simulink model "Non_linear_simulation_r2018b"  (R2026a)
settings: Solver=ode45  StopTime=5  FixedStep=.002  EnableMultiTasking=on
values from neighbouring files (symbols this model uses):
  A_obs = A - L*C    [MA6217_intial.m]    (also in oberver_performance.m; step1.m = A-L*C)
  alphaPlotHandle = plot(inf,inf,'-b','linewidth',2)    [initialiseVisualiser.m]
  armPartPatchHandle = patch(Xt,Yt,Zt,C,'Edgecolor', edgecolor,'facealpha',facealpha,'clipping','off')    [initialiseVisualiser.m]
  armPartVertices = [X(:) Y(:) Z(:) ones(length(X(:)),1)]'    [initialiseVisualiser.m]
  B_obs = [B, L]    [MA6217_intial.m]    (also in oberver_performance.m = [B L]; step1.m = [B L])
  Bp = 0.0024    [AAP5_setup.m]    (also in plant_parameters.m)
  Br = 0.0024    [AAP5_setup.m]    (also in plant_parameters.m)
  C_obs = eye(4)    [MA6217_intial.m]    (also in oberver_performance.m; step1.m)
  D_obs = zeros(4,3)    [MA6217_intial.m]    (also in oberver_performance.m; step1.m)
  drivePartPatchHandle = patch(Xt,Yt,Zt,C,'Edgecolor', edgecolor,'facealpha',facealpha,'clipping','off')    [initialiseVisualiser.m]
  drivePartVertices = [X(:) Y(:) Z(:) ones(length(X(:)),1)]'    [initialiseVisualiser.m]
  eta_g = 0.9    [AAP5_setup.m]    (also in plant_parameters.m)
  eta_m = 0.69    [AAP5_setup.m]    (also in plant_parameters.m)
  frameRate = 50    [AAP5_setup.m]
  G = N4/N5 * N2/N3    (= 70)    [AAP5_setup.m]    (also in oberver_performance.m = [0 0; plant_parameters.m)
  g = 9.81    [AAP5_setup.m]    (also in plant_parameters.m)
  J = Jarm + Jrotor_eff    (= 0.00608016405667)    [AAP5_setup.m]    (also in plant_parameters.m)
  Jp = mp*Lp^2/12    (= 0.00119873080146)    [AAP5_setup.m]    (also in plant_parameters.m)
  K = K_all(selected_case,:)    [lqr_design.m]    (also in step2.m; step3.m = baseline.K; verify_feedforward.m = design.Kx)
  kb = kt    (= 0.00768)    [AAP5_setup.m]    (also in plant_parameters.m)
  kt = 7.68e-3    (= 0.00768)    [AAP5_setup.m]    (also in plant_parameters.m)
  Lp = 0.33655    [AAP5_setup.m]    (also in plant_parameters.m)
  lp = Lp/2    (= 0.168275)    [AAP5_setup.m]    (also in plant_parameters.m)
  mp = 0.127    [AAP5_setup.m]    (also in plant_parameters.m)
  pendPartPatchHandle = patch(Xt,Yt,Zt,C,'Edgecolor', edgecolor,'facealpha',facealpha,'clipping','off')    [initialiseVisualiser.m]
  pendPartVertices = [X(:) Y(:) Z(:) ones(length(X(:)),1)]'    [initialiseVisualiser.m]
  r = 0.2159    [AAP5_setup.m]    (also in plant_parameters.m)
  Ra = 2.6    [AAP5_setup.m]    (also in plant_parameters.m)
  thetaPlotHandle = plot(inf,inf,'-r','linewidth',2)    [initialiseVisualiser.m]
  x0 = [0; deg2rad(5); 0; 0]    [lqr_design.m]    (also in step2.m = [0; 5*pi/180; 0; 0])
settings Model: Creator=Dylan  LastModifiedBy=DELL
settings DataIOCC: SaveFormat=StructureWithTime
settings HardwareCC: ProdHWDeviceType=Specified

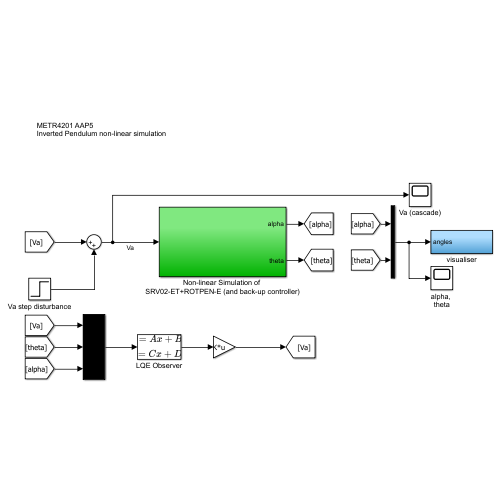
[thumbnail: Simulink's stored preview of the top-level diagram]
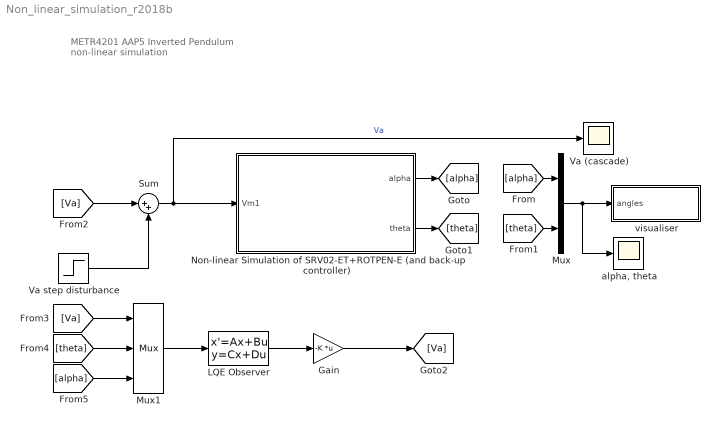
== system Non_linear_simulation_r2018b ==
  note: METR4201 AAP5
      | Inverted Pendulum non-linear simulation
  Gain : Gain  Gain=-K  Multiplication=Matrix(K*u)
  LQE Observer : StateSpace  A=A_obs  B=B_obs  C=C_obs  D=D_obs  InitialCondition=x0
  Mux : Mux  Inputs=2
  Mux1 : Mux  Inputs=3
  Non-linear Simulation of SRV02-ET+ROTPEN-E (and back-up controller) : Subsystem
  Sum : Sum  Inputs=|++
  Va (cascade) : Scope
      settings: ActiveDisplayYMinimum=-0.29963  ActiveDisplayYMaximum=1.44256
  Va step disturbance : Step  FinalValue=0  SampleTime=0
  "alpha, theta" : Scope
      settings: ActiveDisplayYMinimum=-261496.6588  ActiveDisplayYMaximum=29061.54521  DataLoggingVariableName=nonlinear
  visualiser : Subsystem
  wires:
  Mux/1 -> "alpha, theta"/1, visualiser/1(angles)
  Non-linear Simulation of SRV02-ET+ROTPEN-E (and back-up controller)/2(theta) -> [theta]
  Non-linear Simulation of SRV02-ET+ROTPEN-E (and back-up controller)/1(alpha) -> [alpha]
  Sum/1 -> Va (cascade)/1, Non-linear Simulation of SRV02-ET+ROTPEN-E (and back-up controller)/1(Vm1)  "Va"
  Va step disturbance/1 -> Sum/2
  [Va] -> Sum/1
  [theta] -> Mux/2
  [alpha] -> Mux/1
  Mux1/1 -> LQE Observer/1
  [Va] -> Mux1/1
  [theta] -> Mux1/2
  [alpha] -> Mux1/3
  LQE Observer/1 -> Gain/1
  Gain/1 -> [Va]

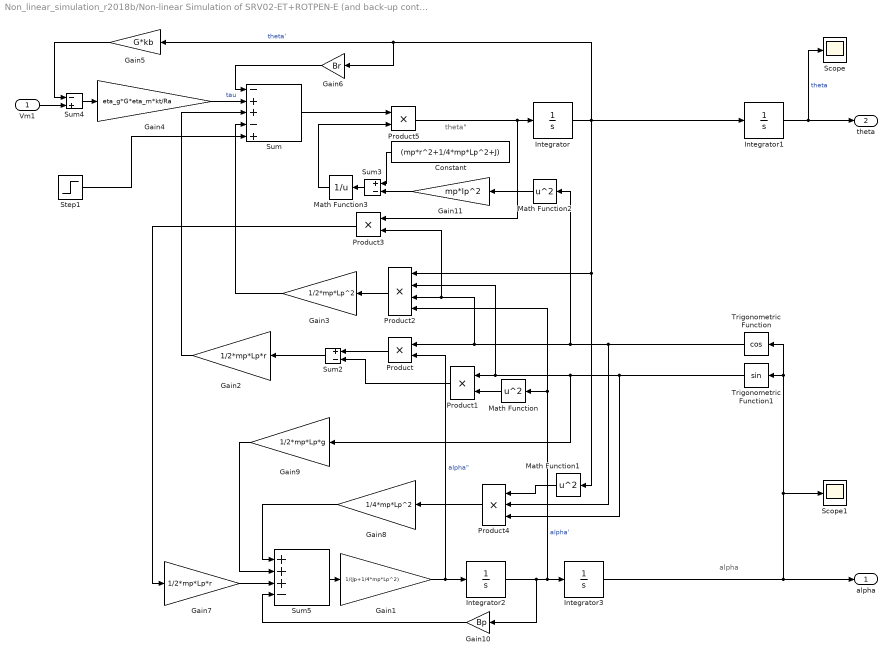
== system Non_linear_simulation_r2018b/Non-linear Simulation of SRV02-ET+ROTPEN-E (and back-up controller) ==
  note: theta"
  note: alpha
  Vm1 : Inport
  Constant : Constant  Value=(mp*r^2+1/4*mp*Lp^2+J)
  Gain1 : Gain  Gain=1/(Jp+1/4*mp*Lp^2)
  Gain10 : Gain  Gain=Bp
  Gain11 : Gain  Gain=mp*lp^2
  Gain2 : Gain  Gain=1/2*mp*Lp*r
  Gain3 : Gain  Gain=1/2*mp*Lp^2
  Gain4 : Gain  Gain=eta_g*G*eta_m*kt/Ra
  Gain5 : Gain  Gain=G*kb
  Gain6 : Gain  Gain=Br
  Gain7 : Gain  Gain=1/2*mp*Lp*r
  Gain8 : Gain  Gain=1/4*mp*Lp^2
  Gain9 : Gain  Gain=1/2*mp*Lp*g
  Integrator : Integrator
  Integrator1 : Integrator
  Integrator2 : Integrator
  Integrator3 : Integrator  InitialCondition=5*pi/180
  Math Function : Math  Operator=square  SignedPower=on
  Math Function1 : Math  Operator=square  SignedPower=on
  Math Function2 : Math  Operator=square  SignedPower=on
  Math Function3 : Math  Operator=reciprocal  SignedPower=on
  Product{,1,3,5} (4 alike) : Product  RndMeth=Zero
  Product2 : Product  Inputs=4  RndMeth=Zero
  Product4 : Product  Inputs=3  RndMeth=Zero
  Scope : Scope
      settings: ActiveDisplayYMinimum=-1  ActiveDisplayYMaximum=1  DataLoggingVariableName=ScopeData3
  Scope1 : Scope
      settings: ActiveDisplayYMinimum=-0.00537  ActiveDisplayYMaximum=0.0023  DataLoggingVariableName=ScopeData4
  Step1 : Step  Time=.1  FinalValue=0  SampleTime=0
  Sum : Sum  Inputs=-++-+
  Sum2 : Sum  Inputs=+-
  Sum3 : Sum  Inputs=+-
  Sum4 : Sum  Inputs=-+
  Sum5 : Sum  Inputs=+++-
  Trigonometric Function : Trigonometry  Operator=cos
  Trigonometric Function1 : Trigonometry
  alpha : Outport  VectorParamsAs1DForOutWhenUnconnected=off
  theta : Outport  Port=2  VectorParamsAs1DForOutWhenUnconnected=off
  wires:
  Product5/1 -> Product3/1, Integrator/1
  Product/1 -> Sum2/1
  Sum2/1 -> Gain2/1
  Sum/1 -> Product5/1
  Gain9/1 -> Sum5/2
  Gain10/1 -> Sum5/4
  Math Function2/1 -> Gain11/1
  Gain11/1 -> Sum3/2
  Constant/1 -> Sum3/1
  Sum3/1 -> Math Function3/1
  Math Function3/1 -> Product5/2
  Sum5/1 -> Gain1/1
  Gain2/1 -> Sum/3
  Gain7/1 -> Sum5/3
  Product3/1 -> Gain7/1
  Trigonometric Function1/1 -> Product4/3, Gain9/1, Product2/2, Product1/1
  Math Function/1 -> Product1/2
  Product1/1 -> Sum2/2
  Product4/1 -> Gain8/1
  Product2/1 -> Gain3/1
  Vm1/1 -> Sum4/2
  Gain5/1 -> Sum4/1
  Sum4/1 -> Gain4/1
  Gain4/1 -> Sum/2  "tau"
  Gain6/1 -> Sum/1
  Gain3/1 -> Sum/4
  Gain8/1 -> Sum5/1
  Math Function1/1 -> Product4/1
  Integrator2/1 -> Gain10/1, Integrator3/1, Math Function/1, Product2/4  "alpha'"
  Gain1/1 -> Product/2, Integrator2/1  "alpha\""
  Trigonometric Function/1 -> Product4/2, Product3/2, Product2/3, Product/1, Math Function2/1
  Integrator/1 -> Math Function1/1, Product2/1, Integrator1/1, Gain6/1, Gain5/1  "theta'"
  Integrator1/1 -> theta/1, Scope/1  "theta"
  Step1/1 -> Sum/5
  Integrator3/1 -> Scope1/1, Trigonometric Function/1, Trigonometric Function1/1, alpha/1

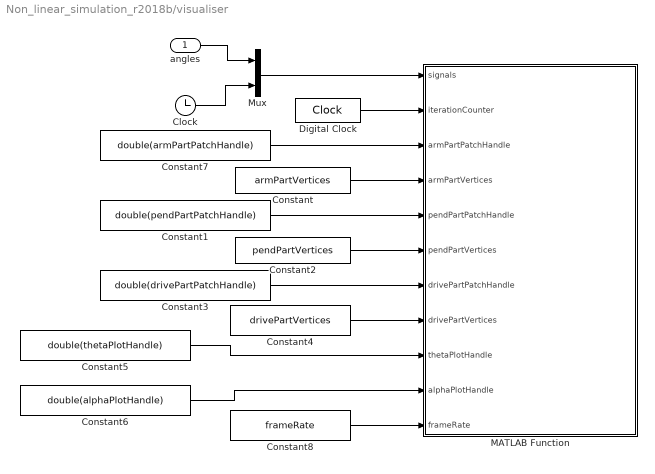
== system Non_linear_simulation_r2018b/visualiser ==
  angles : Inport
  Clock : Clock
  Constant : Constant  Value=armPartVertices  VectorParams1D=off
  Constant1 : Constant  Value=double(pendPartPatchHandle)
  Constant2 : Constant  Value=pendPartVertices  VectorParams1D=off
  Constant3 : Constant  Value=double(drivePartPatchHandle)
  Constant4 : Constant  Value=drivePartVertices  VectorParams1D=off
  Constant5 : Constant  Value=double(thetaPlotHandle)
  Constant6 : Constant  Value=double(alphaPlotHandle)
  Constant7 : Constant  Value=double(armPartPatchHandle)
  Constant8 : Constant  Value=frameRate  VectorParams1D=off
  Digital Clock : DigitalClock  SampleTime=.001
  MATLAB Function : MATLAB Function  TreatAsAtomicUnit=on
  Mux : Mux  Inputs=2
  wires:
  angles/1 -> Mux/1
  Mux/1 -> MATLAB Function/1(signals)
  Clock/1 -> Mux/2
  Constant7/1 -> MATLAB Function/3(armPartPatchHandle)
  Constant/1 -> MATLAB Function/4(armPartVertices)
  Constant1/1 -> MATLAB Function/5(pendPartPatchHandle)
  Constant2/1 -> MATLAB Function/6(pendPartVertices)
  Constant6/1 -> MATLAB Function/10(alphaPlotHandle)
  Constant5/1 -> MATLAB Function/9(thetaPlotHandle)
  Constant4/1 -> MATLAB Function/8(drivePartVertices)
  Constant3/1 -> MATLAB Function/7(drivePartPatchHandle)
  Digital Clock/1 -> MATLAB Function/2(iterationCounter)
  Constant8/1 -> MATLAB Function/11(frameRate)

== matlab function Non_linear_simulation_r2018b/visualiser/MATLAB Function ==
  data: signals input; iterationCounter input; armPartPatchHandle input; armPartVertices input; pendPartPatchHandle input; pendPartVertices input; drivePartPatchHandle input; drivePartVertices input; thetaPlotHandle input; alphaPlotHandle input; frameRate input
function  updateVisualiser(signals, iterationCounter, armPartPatchHandle, armPartVertices, pendPartPatchHandle, pendPartVertices, drivePartPatchHandle, drivePartVertices, thetaPlotHandle, alphaPlotHandle, frameRate)

%
% We need the set and get functions for changing plots.
%
coder.extrinsic('set');
coder.extrinsic('get');


%
% Clear the theta and alpha plots if this is the first iteration.
%
if iterationCounter == 0
    set(thetaPlotHandle,'xData',inf,'yData',inf);
    set(alphaPlotHandle,'xData',inf,'yData',inf);
end

%
% Only update figure on every 2nd iteration.
%
if mod(iterationCounter,1/frameRate) == 0
    
    alphaAngle = signals(1);
    thetaAngle = signals(2);
    currentTime = signals(3);
    
    %
    % New frame transformations.
    %
    BaseToArm = homogeneous_func(0,0,thetaAngle,0,0,12e-2);
    ArmToPendulum = homogeneous_func(alphaAngle,0,0,14.2e-2,0,5e-2);
    BaseToDrive = homogeneous_func(0,0,(-thetaAngle*5),0,0.036,12e-2);
    
    %
    % Update arm parts.
    %
    armPart_vertices_G_frame = BaseToArm * armPartVertices;
    Xt = reshape(armPart_vertices_G_frame(1,:),3,[]);
    Yt = reshape(armPart_vertices_G_frame(2,:),3,[]);
    Zt = reshape(armPart_vertices_G_frame(3,:),3,[]);
    set(armPartPatchHandle, 'xData', Xt, 'yData', Yt, 'zData', Zt);
    
    %
    % Update pendulum parts.
    %
    pendPart_vertices_G_frame = BaseToArm * ArmToPendulum* pendPartVertices;
    Xt = reshape(pendPart_vertices_G_frame(1,:),3,[]);
    Yt = reshape(pendPart_vertices_G_frame(2,:),3,[]);
    Zt = reshape(pendPart_vertices_G_frame(3,:),3,[]);
    set(pendPartPatchHandle, 'xData', Xt, 'yData', Yt, 'zData', Zt);
    
    %
    % Update drive gear parts.
    %
    drivePart_vertices_G_frame = BaseToDrive* drivePartVertices;
    Xt = reshape(drivePart_vertices_G_frame(1,:),3,[]);
    Yt = reshape(drivePart_vertices_G_frame(2,:),3,[]);
    Zt = reshape(drivePart_vertices_G_frame(3,:),3,[]);
    set(drivePartPatchHandle, 'xData', Xt, 'yData', Yt, 'zData', Zt);
    
    %
    % Update theta plot.
    %
    times = [get(thetaPlotHandle,'xData'), currentTime];
    thetaAngles = [get(thetaPlotHandle,'yData'), thetaAngle*180/pi];
    set(thetaPlotHandle,'xdata',times,'ydata',thetaAngles);
    
    %
    % Update alpha plot.
    %
    times = [get(alphaPlotHandle,'xData'), currentTime];
    alphaAngles = [get(alphaPlotHandle,'yData'), alphaAngle*180/pi];
    set(alphaPlotHandle,'xdata',times,'ydata',alphaAngles);
end
end

function [T] = homogeneous_func(ROLL, PITCH, YAW, X, Y, Z)
T=zeros(4,4);
T(1,1) = cos(YAW)*cos(PITCH);
T(1,2) = cos(YAW)*sin(PITCH)*sin(ROLL)-sin(YAW)*cos(ROLL);
T(1,3) = cos(YAW)*sin(PITCH)*cos(ROLL)+sin(YAW)*sin(ROLL);
T(1,4) = X;
T(2,1) = sin(YAW)*cos(PITCH);
T(2,2) = sin(YAW)*sin(PITCH)*sin(ROLL)+cos(YAW)*cos(ROLL);
T(2,3) = sin(YAW)*sin(PITCH)*cos(ROLL)-cos(YAW)*sin(ROLL);
T(2,4) = Y;
T(3,1) = -sin(PITCH);
T(3,2) = cos(PITCH)*sin(ROLL);
T(3,3) = cos(PITCH)*cos(ROLL);
T(3,4) = Z;
T(4,4) = 1;
end
